simulink model "hybridpsversion21a"  (R2024a)
settings: Solver=VariableStepAuto  StartTime=0.0  StopTime=5  RelTol=1e-3
undefined symbols (not defined in the file): Ion, Lithium
libraries: spsSeriesRLCBranchLib x8, spsGroundLib x4, spsMosfetLib x4, spsDiodeLib x3, spsBatteryLib x1, spsPVArrayLib x1, spsPermanentMagnetSynchronousMachineLib x1, spsUniversalBridgeLib x1, spsVoltageMeasurementLib x1, spspowerguiLib x1
settings Model: Creator=sarve  LastModifiedBy=Aswin

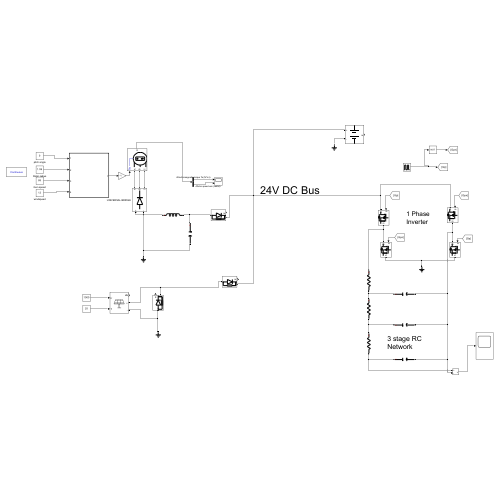
[thumbnail: Simulink's stored preview of the top-level diagram]
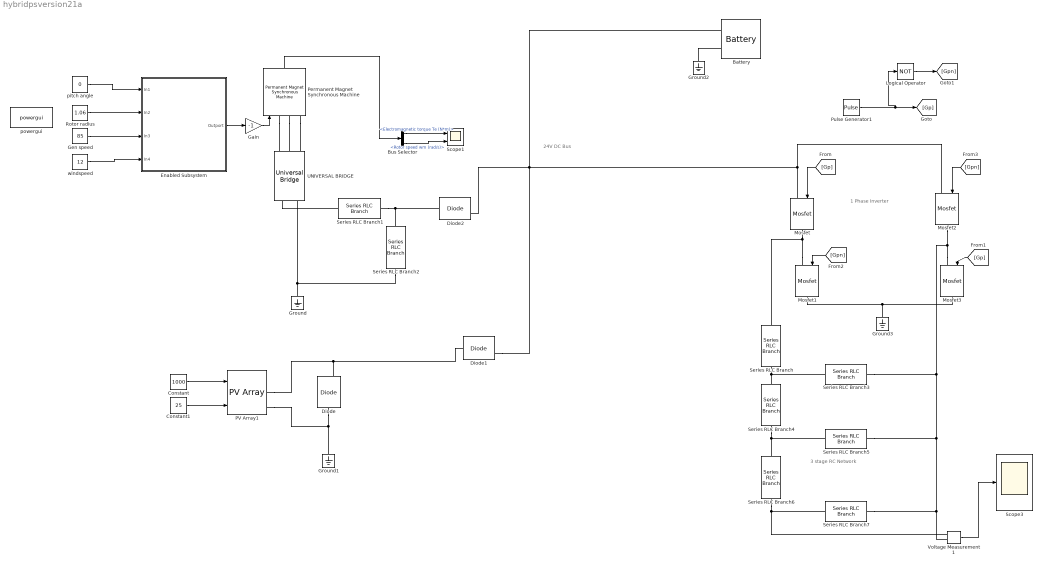
== system hybridpsversion21a ==
  note: 3 stage RC
      | Network
  note: 24V DC Bus
  note: 1 Phase
      | Inverter
  Battery : spsBatteryLib/Battery  BatType=Lithium-Ion  NomV=24  NomQ=15  SOC=50  Batt_Tr=30  PresetModel=on  MaxQ=15  MinV=18  FullV=27.9357  Dis_rate=6.5217  R=0.016  Normal_OP=13.5652  expZone="[25.9293     0.736957]"
  Bus Selector : BusSelector  OutputSignals=Electromagnetic torque Te (N*m),Rotor speed wm (rad/s)
  Constant : Constant  Value=1000
  Constant1 : Constant  Value=25
  Diode : spsDiodeLib/Diode  Ron=0.001  Lon=0  Vf=0.8  IC=0  UseSnubber=0  Rs=500  Cs=250e-9  Measurements=on
  Diode1 : spsDiodeLib/Diode  Ron=0.001  Lon=0  Vf=0.8  IC=0  UseSnubber=0  Rs=500  Cs=250e-9  Measurements=on
  Diode2 : spsDiodeLib/Diode  Ron=0.001  Lon=0  Vf=0.8  IC=0  UseSnubber=0  Rs=500  Cs=250e-9  Measurements=on
  Enabled Subsystem : Subsystem  TreatAsAtomicUnit=on
  Gain : Gain  Gain=-1
  Gen speed : Constant  Value=85
  Ground{,1..3} (4 alike) : spsGroundLib/Ground  LConnTagsString=a
  Logical Operator : Logic  Operator=NOT  AllPortsSameDT=off  OutDataTypeStr=boolean
  Mosfet{,1..3} (4 alike) : spsMosfetLib/Mosfet  Ron=0.1  Lon=0  Rd=0.01  Vfd=0  IC=0  Rs=1e5  Cs=inf  Measurements=off
  PV Array1 : spsPVArrayLib/PV Array  Npar=40  Nser=1  PlotType=array @ 1000 W/m2 & specified temperatures  S_vec="[ 1000  500  100 ]"  Temp_C_vec="[ 45 25  ]"  ModuleName=User-defined  PlotWhenSelected=off  Pm=45  Ncell=36  Voc=25.35  Isc=2.4  Vm=20  Im=2.25  beta_Voc_pc=-0.3  alpha_Isc_pc=0  beta_Voc=-0.07605  alpha_Isc=0  IL=2.415  I0=7.5435e-12  nI=1.0355  Rsh=457.6706  Rs=1.1136  RobustModel=off  RobustCellTemperature=313.3991  BAL=on  Tc=1e-6  Tfilter=5e-5
  Permanent Magnet Synchronous Machine : spsPermanentMagnetSynchronousMachineLib/Permanent Magnet Synchronous Machine  NbPhases=3  FluxDistribution=Sinusoidal  RotorType=Round  MechanicalLoad=Torque Tm  PresetModel=No  ShowDetailedParameters=on  MeasurementBus=off  Resistance=0.0485  Inductance=8.5e-3  dqInductances=[8.5e-3,8.5e-3]  La=0.000395  MachineConstant=Flux linkage established by magnets (V.s)  Flux=0.1194  VoltageCst=86.6271  TorqueCst=0.7164  Flat=120  Mechanical=[0.0027 0.0004924 4 0]  PolePairs=4  InitialConditions=[0,0, 0,0]  InitialConditions5ph=[0 0 0 0 0 0]  RefAngle=90 degrees behind phase A axis (modified Park)  IterativeDiscreteModel=Trapezoidal non iterative  TsBlock=-1  TsPowergui=0
  Pulse Generator1 : DiscretePulseGenerator  PulseType=Time based  Period=0.01  PulseWidth=50
  Rotor radius : Constant  Value=1.06
  Scope1 : Scope  NumInputPorts=2
  Scope3 : Scope
  Series RLC Branch : spsSeriesRLCBranchLib/Series RLC Branch  LConnTagsString=__new0  RConnTagsString=__new0  BranchType=R  Resistance=10  Inductance=1e-3  SetiL0=off  InitialCurrent=0  Capacitance=1e-6  Setx0=off  InitialVoltage=0  Measurements=None
  Series RLC Branch1 : spsSeriesRLCBranchLib/Series RLC Branch  LConnTagsString=__new0  RConnTagsString=__new0  BranchType=L  Resistance=1  Inductance=1.1e-3  SetiL0=off  InitialCurrent=0  Capacitance=1e-6  Setx0=off  InitialVoltage=0  Measurements=None
  Series RLC Branch2 : spsSeriesRLCBranchLib/Series RLC Branch  LConnTagsString=__new0  RConnTagsString=__new0  BranchType=C  Resistance=1  Inductance=1e-3  SetiL0=off  InitialCurrent=0  Capacitance=23e-6  Setx0=off  InitialVoltage=0  Measurements=None
  Series RLC Branch3 : spsSeriesRLCBranchLib/Series RLC Branch  LConnTagsString=__new0  RConnTagsString=__new0  BranchType=C  Resistance=100e3  Inductance=1e-3  SetiL0=off  InitialCurrent=0  Capacitance=4.7e-5  Setx0=off  InitialVoltage=0  Measurements=None
  Series RLC Branch4 : spsSeriesRLCBranchLib/Series RLC Branch  LConnTagsString=__new0  RConnTagsString=__new0  BranchType=R  Resistance=10  Inductance=1e-3  SetiL0=off  InitialCurrent=0  Capacitance=1e-6  Setx0=off  InitialVoltage=0  Measurements=None
  Series RLC Branch5 : spsSeriesRLCBranchLib/Series RLC Branch  LConnTagsString=__new0  RConnTagsString=__new0  BranchType=C  Resistance=100e3  Inductance=1e-3  SetiL0=off  InitialCurrent=0  Capacitance=4.7e-5  Setx0=off  InitialVoltage=0  Measurements=None
  Series RLC Branch6 : spsSeriesRLCBranchLib/Series RLC Branch  LConnTagsString=__new0  RConnTagsString=__new0  BranchType=R  Resistance=10  Inductance=1e-3  SetiL0=off  InitialCurrent=0  Capacitance=1e-6  Setx0=off  InitialVoltage=0  Measurements=None
  Series RLC Branch7 : spsSeriesRLCBranchLib/Series RLC Branch  LConnTagsString=__new0  RConnTagsString=__new0  BranchType=C  Resistance=100e3  Inductance=1e-3  SetiL0=off  InitialCurrent=0  Capacitance=4.7e-5  Setx0=off  InitialVoltage=0  Measurements=None
  UNIVERSAL BRIDGE : spsUniversalBridgeLib/Universal Bridge  Arms=3  SnubberResistance=100  SnubberCapacitance=0.1e-6  Device=Diodes  Ron=1e-3  Lon=0  ForwardVoltages="[  0  0  ]"  ForwardVoltage=0.8  GTOparameters=[ 10e-6 , 20e-6 ]  IGBTparameters=[ 1e-6 , 2e-6 ]  Measurements=Device currents  Measurements_2=None  converterType=Rectifier
  Voltage Measurement1 : spsVoltageMeasurementLib/Voltage Measurement  PhasorSimulation=off  OutputType=Complex  PSBequivalent=0
  pitch angle : Constant  Value=0
  powergui : spspowerguiLib/powergui  Priority=1  SimulationMode=Continuous  SampleTime=2e-6  frequency=60  Iterations=50  frequencyindice=0  Pbase=100e6  ErrMax=1e-4  UnitsV=kV  UnitsW=MW  buscounter=0  FunctionMessages=off  echomessages=off  EnableUseOfTLC=off  CurrentSourceSwitches=off  DisableSnubberDevices=off  DisableRonSwitches=off  DisableVfSwitches=off  DisplayEquations=off  AutomaticDiscreteSolvers=off  SolverType=Tustin/Backward Euler (TBE)  Interpol=off  ExternalGateDelay=off  methode=off  Ts=100  x0status=blocks  SPID=on  SwTol=0  HookPort=off  NonlinearTolerance=1e-4  nMaxIteration=100  ContinueOnMaxIteration=off  RestoreLinks=warning  ResistiveCurrentMeasurement=off  Frange=[0:2:500]  Ylog=off  Xlog=on  ShowGrid=off  save=off  variable=ZData  structure=0  ZoomFFT=off  StartTime=0.0  cycles=1  DisplayStyle=1  fundamental=60  FreqAxis=off  MaxFrequency=1000  frequencyindicesteady=1  RmsSteady=1  display=off
  windspeed : Constant  Value=12
  wires:
  Permanent Magnet Synchronous Machine/1 -> Bus Selector/1
  Bus Selector/1 -> Scope1/1  "<Electromagnetic torque Te (N*m)>"
  Bus Selector/2 -> Scope1/2  "<Rotor speed wm (rad/s)>"
  pitch angle/1 -> Enabled Subsystem/1(In1)
  Rotor radius/1 -> Enabled Subsystem/2(In2)
  Gen speed/1 -> Enabled Subsystem/3(In3)
  windspeed/1 -> Enabled Subsystem/4(In4)
  Enabled Subsystem/1(Outport) -> Gain/1
  Gain/1 -> Permanent Magnet Synchronous Machine/1
  Constant1/1 -> PV Array1/2
  Constant/1 -> PV Array1/1
  Pulse Generator1/1 -> [Gp], Logical Operator/1
  Voltage Measurement1/1 -> Scope3/1
  [Gp] -> Mosfet/1
  [Gp] -> Mosfet3/1
  Logical Operator/1 -> [Gpn]
  [Gpn] -> Mosfet1/1
  [Gpn] -> Mosfet2/1
  connections:
  Series RLC Branch1/RConn1 -- Series RLC Branch2/LConn1 -- Diode2/LConn1
  Series RLC Branch2/RConn1 -- Ground/LConn1 -- UNIVERSAL BRIDGE/RConn2
  Permanent Magnet Synchronous Machine/LConn1 -- UNIVERSAL BRIDGE/LConn1
  Permanent Magnet Synchronous Machine/LConn2 -- UNIVERSAL BRIDGE/LConn2
  Permanent Magnet Synchronous Machine/LConn3 -- UNIVERSAL BRIDGE/LConn3
  UNIVERSAL BRIDGE/RConn1 -- Series RLC Branch1/LConn1
  Diode/LConn1 -- Ground1/LConn1 -- PV Array1/RConn2
  PV Array1/RConn1 -- Diode1/LConn1 -- Diode/RConn1
  Mosfet/LConn1 -- Mosfet2/LConn1 -- Diode1/RConn1 -- Diode2/RConn1 -- Battery/LConn1
  Ground2/LConn1 -- Battery/LConn2
  Mosfet3/LConn1 -- Voltage Measurement1/LConn2 -- Series RLC Branch7/RConn1 -- Series RLC Branch5/RConn1 -- Series RLC Branch3/RConn1 -- Mosfet2/RConn1
  Mosfet1/LConn1 -- Mosfet/RConn1 -- Series RLC Branch/LConn1
  Series RLC Branch/RConn1 -- Series RLC Branch3/LConn1 -- Series RLC Branch4/LConn1
  Series RLC Branch4/RConn1 -- Series RLC Branch5/LConn1 -- Series RLC Branch6/LConn1
  Series RLC Branch6/RConn1 -- Series RLC Branch7/LConn1 -- Voltage Measurement1/LConn1
  Ground3/LConn1 -- Mosfet1/RConn1 -- Mosfet3/RConn1

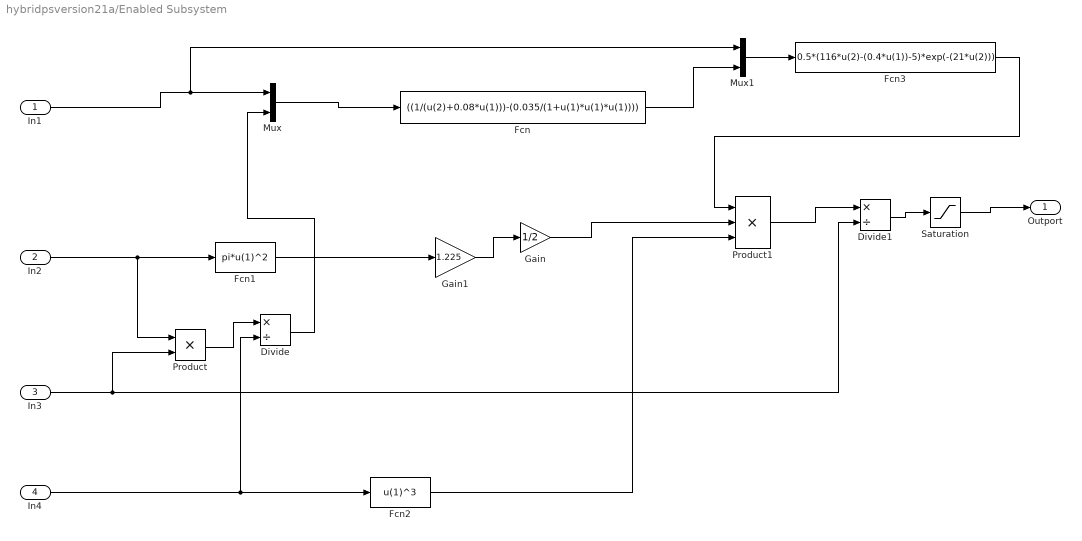
== system hybridpsversion21a/Enabled Subsystem ==
  In1 : Inport
  In2 : Inport  Port=2
  In3 : Inport  Port=3
  In4 : Inport  Port=4
  Divide : Product  Inputs=*/
  Divide1 : Product  Inputs=*/
  Fcn : Fcn  Expr=((1/(u(2)+0.08*u(1)))-(0.035/(1+u(1)*u(1)*u(1))))
  Fcn1 : Fcn  Expr=pi*u(1)^2
  Fcn2 : Fcn  Expr=u(1)^3
  Fcn3 : Fcn  Expr=0.5*(116*u(2)-(0.4*u(1))-5)*exp(-(21*u(2)))
  Gain : Gain  Gain=1/2
  Gain1 : Gain  Gain=1.225
  Mux : Mux  Inputs=2
  Mux1 : Mux  Inputs=2
  Product : Product
  Product1 : Product  Inputs=3
  Saturation : Saturate  UpperLimit=inf  LowerLimit=1e-2
  Outport : Outport
  wires:
  In2/1 -> Fcn1/1, Product/1
  In3/1 -> Divide1/2, Product/2
  Product/1 -> Divide/1
  In1/1 -> Mux1/1, Mux/1
  Divide/1 -> Mux/2
  Mux/1 -> Fcn/1
  In4/1 -> Divide/2, Fcn2/1
  Fcn/1 -> Mux1/2
  Mux1/1 -> Fcn3/1
  Fcn3/1 -> Product1/1
  Fcn2/1 -> Product1/3
  Gain/1 -> Product1/2
  Gain1/1 -> Gain/1
  Fcn1/1 -> Gain1/1
  Product1/1 -> Divide1/1
  Divide1/1 -> Saturation/1
  Saturation/1 -> Outport/1
